simulink model "ball_balance_cl"  (R2026b)
settings: Solver=daessc  StopTime=bb.ref.T  MaxStep=1e-3
PreLoadFcn:
  | addpath(fileparts(which(bdroot))); bb = bb_params();
InitFcn:
  | addpath(fileparts(which(bdroot))); bb = bb_params();
values from neighbouring files (symbols this model uses):
  bb = bb_params();',      'Solver', 'daessc', 'StopTime', stopTime, 'MaxStep', '1e-3',      'RelTol', '1e-3', 'SaveOutput', 'on', 'SaveFormat', 'Dataset',      'ReturnWorkspaceOutputs', 'on', 'SignalLogging', 'on')    [build_bb_model.m]    (also in design_controller.m = bb_params(); run_closed_loop.m = bb_params(); run_open_loop_test.m = bb_params())
  deg = 90    [build_bb_model.m]
  kg = blk(C, 'simulink/Math Operations/Gain', 'LQI Gain', [860 100])    [build_bb_model.m]
  s = @(t0, T) min(max((t - t0)/T, 0), 1)    [bb_params.m]    (also in run_open_loop_test.m = squeeze(srv.Data); if size(s,1) == 2 && size(s,2) ~= 2, s = )
undefined symbols (not defined in the file or in its folder): DiscIntNeverNeededParam, X, Y, Z
libraries: sm_lib x54, nesl_utility x9
(part 1 of 2)
settings Model: Creator=PC  LastModifiedBy=PC
settings SimscapeCC: SimscapeLogType=all  SimscapeNominalValues="[{\"value\":\"1\",\"unit\":\"A\"},{\"value\":\"1\",\"unit\":\"bar\"},{\"value\":\"1\",\"unit\":\"cm^2\"},{\"value\":\"1\",\"unit\":\"cm^3/s\"},{\"value\":\"1\",\"unit\":\"kJ/kg\"},{\"value\":\"1\",\"unit\":\"kW\"},{\"value\":\"1\",\"unit\":\"l\"},{\"value\":\"1\",\"unit\":\"N\"},{\"value\":\"1\",\"unit\":\"N*m\"},{\"value\":\"1\",\"unit\":\"V\"},{\"value\":\"0.001\",\"unit\":\"Wb\"}]"  SimscapeUseEnergyAccounting=off

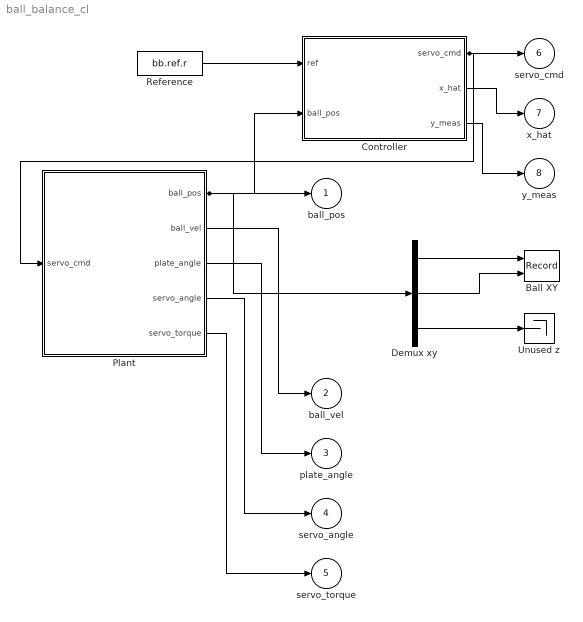
== system ball_balance_cl ==
  Ball XY : Record  NumPorts=2.0  FileSettingsInternal="{\"entries\":[{\"content\":{\"excelSettings\":{\"content\":{},\"type\":\"Streamout.ExcelSettings\"},\"parquetSettings\":{\"content\":{},\"type\":\"Streamout.ParquetSettings\"}},\"type\":\"Streamout.FileSettingStorage\",\"uuid\":\"\"}],\"packageUris\":[\"http:\\/\\/schema.mathworks.com\\/mf0\\/streamout_blocks\\/R2020a\"],\"version\":\"1.0\"}"  FrameSettings=[0, 0]  Layout=[1 1]  SignalsInternal="{\"entries\":[{\"content\":{\"signals\":[{\"content\":{\"blockPath\":[],\"dimensions\":[1],\"domain\":\"\",\"lineColor\":\"#a2142f\",\"plots\":[ 1 ],\"port\":1,\"signalID\":1,\"signalName\":\"XY Graph:1\"},\"type\":\"RecordBlkView.Signal\",\"uuid\":\"\"},{\"content\":{\"blockPath\":[],\"dimensions\":[1],\"domain\":\"\",\"lineColor\":\"#139fff\",\"plots\":[ 1 ],\"port\":2,\"signalID\":2,\"signalName\":\"XY Graph:2\"},\"type\":\"RecordBlkView.Signal\",\"uuid\":\"\"}]},\"type\":\"RecordBlkView.InputSignals\",\"uuid\":\"\"}],\"packageUris\":[\"http:\\/\\/schema.mathworks.com\\/mf0\\/streamout_blocks\\/R2020a\"],\"version\":\"1.0\"}"  VisualizationBindings="{\"xyplotplugin\":{\"info\":[{\"series\":[{\"bindingParametersList\":[{\"parameter\":\"X-Axis\",\"signalID\":1,\"signalName\":\"XY Graph:1\"},{\"parameter\":\"Y-Axis\",\"signalID\":2,\"signalName\":\"XY Graph:2\"}],\"seriesID\":0}],\"subplotID\":1}]}}"  CompatibilityTag=XY
  Controller : Subsystem
  Demux xy : Demux  Outputs=3
  Plant : Subsystem
  Reference : FromWorkspace  VariableName=bb.ref.r  OutputAfterFinalValue=Holding final value
  Unused z : Terminator
  ball_pos : Outport
  ball_vel : Outport  Port=2
  plate_angle : Outport  Port=3
  servo_angle : Outport  Port=4
  servo_torque : Outport  Port=5
  servo_cmd : Outport  Port=6
  x_hat : Outport  Port=7
  y_meas : Outport  Port=8
  wires:
  Reference/1 -> Controller/1(ref)
  Controller/2(x_hat) -> x_hat/1
  Plant/1(ball_pos) -> Controller/2(ball_pos), ball_pos/1, Demux xy/1
  Controller/1(servo_cmd) -> Plant/1(servo_cmd), servo_cmd/1
  Plant/2(ball_vel) -> ball_vel/1
  Plant/3(plate_angle) -> plate_angle/1
  Plant/5(servo_torque) -> servo_torque/1
  Plant/4(servo_angle) -> servo_angle/1
  Controller/3(y_meas) -> y_meas/1
  Demux xy/1 -> Ball XY/1
  Demux xy/2 -> Ball XY/2
  Demux xy/3 -> Unused z/1

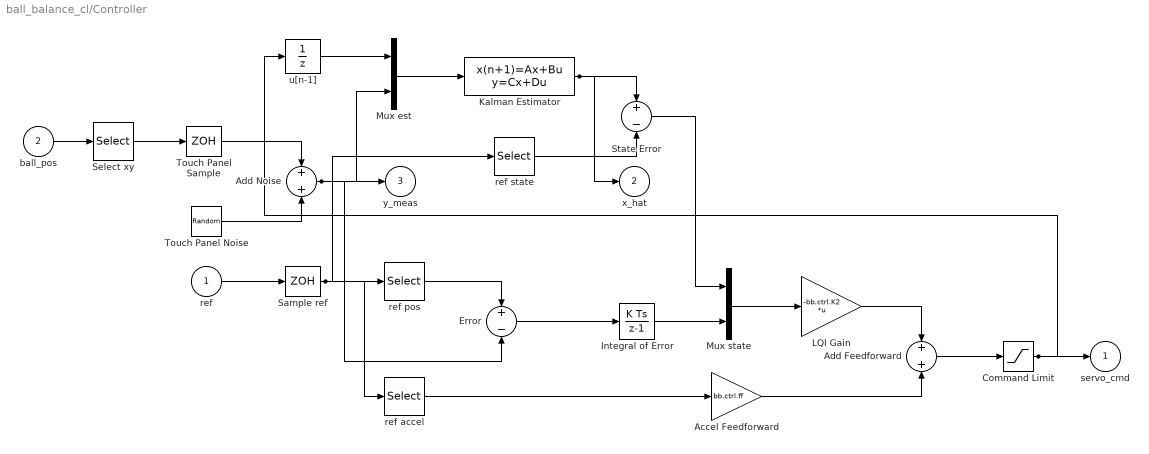
== system ball_balance_cl/Controller ==
  ref : Inport
  ball_pos : Inport  Port=2
  Accel Feedforward : Gain  Gain=bb.ctrl.ff
  Add Feedforward : Sum
  Add Noise : Sum
  Command Limit : Saturate  UpperLimit=bb.ctrl.u_sat  LowerLimit=-bb.ctrl.u_sat
  Error : Sum  Inputs=+-
  Integral of Error : DiscreteIntegrator  gainval=1  SampleTime=bb.ctrl.Ts  LimitOutput=on  UpperSaturationLimit=bb.ctrl.xi_max  LowerSaturationLimit=-bb.ctrl.xi_max  ICPrevOutput=DiscIntNeverNeededParam  ICPrevScaledInput=DiscIntNeverNeededParam
  Kalman Estimator : DiscreteStateSpace  A=bb.ctrl.est2.A  B=bb.ctrl.est2.B  C=bb.ctrl.est2.C  D=bb.ctrl.est2.D  InitialCondition=bb.ctrl.est2.x0  SampleTime=bb.ctrl.Ts
  LQI Gain : Gain  Gain=-bb.ctrl.K2  Multiplication=Matrix(K*u)
  Mux est : Mux  Inputs=2
  Mux state : Mux  Inputs=2
  Sample ref : ZeroOrderHold  SampleTime=bb.ctrl.Ts
  Select xy : Selector  InputPortWidth=3  IndexOptions=Index vector (dialog)  Indices=[1 2]  OutputSizes=1
  State Error : Sum  Inputs=+-
  Touch Panel Noise : RandomNumber  Mean=[0 0]  Variance=(bb.ctrl.noise_on*bb.ctrl.noise_sd)^2*[1 1]  Seed=[11 23]  SampleTime=bb.ctrl.Ts
  Touch Panel Sample : ZeroOrderHold  SampleTime=bb.ctrl.Ts
  ref accel : Selector  InputPortWidth=6  IndexOptions=Index vector (dialog)  Indices=[5 6]  OutputSizes=1
  ref pos : Selector  InputPortWidth=6  IndexOptions=Index vector (dialog)  Indices=[1 2]  OutputSizes=1
  ref state : Selector  InputPortWidth=6  IndexOptions=Index vector (dialog)  Indices=[1 3 2 4]  OutputSizes=1
  u[n-1] : UnitDelay  InitialCondition=[0;0]  SampleTime=bb.ctrl.Ts
  servo_cmd : Outport
  x_hat : Outport  Port=2
  y_meas : Outport  Port=3
  wires:
  ball_pos/1 -> Select xy/1
  Select xy/1 -> Touch Panel Sample/1
  u[n-1]/1 -> Mux est/1
  Touch Panel Sample/1 -> Add Noise/1
  Touch Panel Noise/1 -> Add Noise/2
  Sample ref/1 -> ref state/1, ref pos/1, ref accel/1
  Add Noise/1 -> Error/2, y_meas/1, Mux est/2
  ref/1 -> Sample ref/1
  Mux est/1 -> Kalman Estimator/1
  ref pos/1 -> Error/1
  ref accel/1 -> Accel Feedforward/1
  Kalman Estimator/1 -> State Error/1, x_hat/1
  ref state/1 -> State Error/2
  Error/1 -> Integral of Error/1
  State Error/1 -> Mux state/1
  Integral of Error/1 -> Mux state/2
  Mux state/1 -> LQI Gain/1
  Accel Feedforward/1 -> Add Feedforward/2
  LQI Gain/1 -> Add Feedforward/1
  Add Feedforward/1 -> Command Limit/1
  Command Limit/1 -> u[n-1]/1, servo_cmd/1
